simulink model "permanent_magnet_synchronous_machine"  (R2026b)
settings: Solver=VariableStepAuto
libraries: nesl_utility x24, fl_lib x1, pmsm_uvw_with_harmonics_lib x1
settings Model: Creator=dbagn  LastModifiedBy=d.bagnara

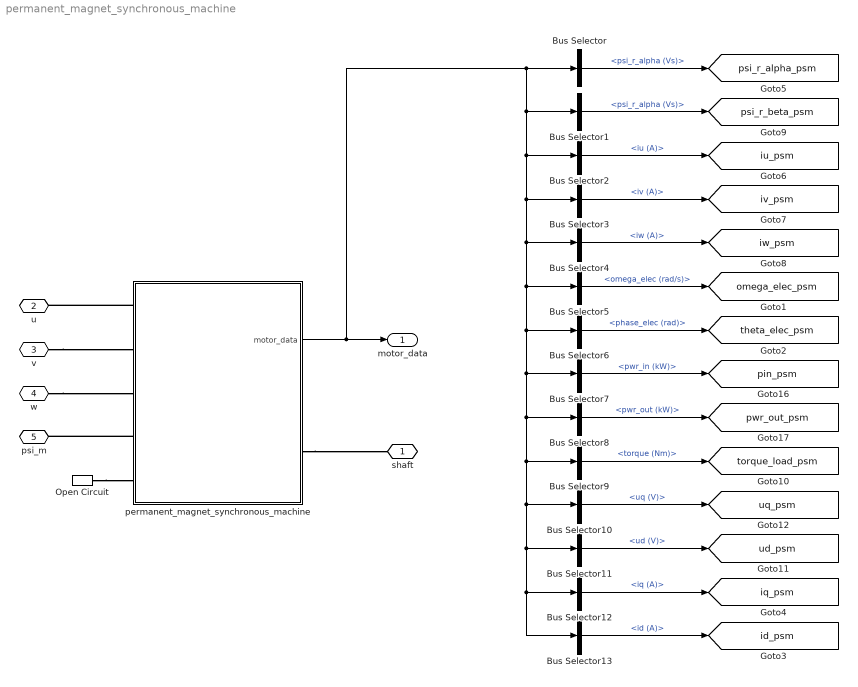
== system permanent_magnet_synchronous_machine ==
  Bus Selector : BusSelector  OutputSignals=psi_r_alpha (Vs)
  Bus Selector1 : BusSelector  OutputSignals=psi_r_alpha (Vs)
  Bus Selector10 : BusSelector  OutputSignals=uq (V)
  Bus Selector11 : BusSelector  OutputSignals=ud (V)
  Bus Selector12 : BusSelector  OutputSignals=iq (A)
  Bus Selector13 : BusSelector  OutputSignals=id (A)
  Bus Selector2 : BusSelector  OutputSignals=iu (A)
  Bus Selector3 : BusSelector  OutputSignals=iv (A)
  Bus Selector4 : BusSelector  OutputSignals=iw (A)
  Bus Selector5 : BusSelector  OutputSignals=omega_elec (rad/s)
  Bus Selector6 : BusSelector  OutputSignals=phase_elec (rad)
  Bus Selector7 : BusSelector  OutputSignals=pwr_in (kW)
  Bus Selector8 : BusSelector  OutputSignals=pwr_out (kW)
  Bus Selector9 : BusSelector  OutputSignals=torque (Nm)
  Open Circuit : fl_lib/Electrical/Electrical Elements/Open Circuit  v_specify=off  v_priority=None  v=0 V  v_nominal_specify=off  v_nominal_value=1  v_nominal_unit=V
  permanent_magnet_synchronous_machine : Subsystem  mask{pp=52, psi_m=3.85, Lmu=5e-6, La=4.6e-3, Lb=4.4e-3, Rs=31.5e-3, Jm=1968, b_linear=0, b_quadratic=0, h5_percent=0, h7_percent=0, psi_r_u_init=0, psi_r_v_init=0, psi_r_w_init=0, omega_init=0, phase_init=0, angle_error=0}
      mask prompts: pp "pole pairs"; psi_m "magnet flux - PsiM (Vs)"; Lmu "Leakage inductance - Lsigma (H)"; La "Phase self inductance - La (H)"; Lb "Phase mutual inductance - Lb (H)"; Rs "Phase resistance - Rs (Ohm)"; Jm "Shaft moment of inertia - Jm (kgm^2)"; b_linear "Linear viscosity - bm (Nms/rad)"; b_quadratic "Quadratic viscosity - bs (Nms^2/rad^2))"; h5_percent "Torque ripple H5 - (percent)"; h7_percent "Torque ripple H7 - (percent)"; psi_r_u_init "Rotor Flux init U - (Vs)"; psi_r_v_init "Rotor Flux init V - (Vs)"; psi_r_w_init "Rotor Flux init W - (Vs)"; omega_init "Rotor Speed init (rad/s)"; phase_init "Rotor Position init (rad)"; angle_error "Angle Error (rad)"
  shaft : PMIOPort  Side=Right
  u : PMIOPort  Port=2  Side=Left
  v : PMIOPort  Port=3  Side=Left
  w : PMIOPort  Port=4  Side=Left
  psi_m : PMIOPort  Port=5  Side=Left
  motor_data : Outport
  tag scope: id_psm=global, iq_psm=global, iu_psm=global, iv_psm=global, iw_psm=global, omega_elec_psm=global, pin_psm=global, psi_r_alpha_psm=global, psi_r_beta_psm=global, pwr_out_psm=global, theta_elec_psm=global, torque_load_psm=global, ud_psm=global, uq_psm=global
  wires:
  Bus Selector11/1 -> [ud_psm]  "<ud (V)>"
  Bus Selector9/1 -> [torque_load_psm]  "<torque (Nm)>"
  Bus Selector12/1 -> [iq_psm]  "<iq (A)>"
  Bus Selector13/1 -> [id_psm]  "<id (A)>"
  Bus Selector1/1 -> [psi_r_beta_psm]  "<psi_r_alpha (Vs)>"
  Bus Selector5/1 -> [omega_elec_psm]  "<omega_elec (rad/s)>"
  Bus Selector4/1 -> [iw_psm]  "<iw (A)>"
  Bus Selector2/1 -> [iu_psm]  "<iu (A)>"
  Bus Selector3/1 -> [iv_psm]  "<iv (A)>"
  Bus Selector6/1 -> [theta_elec_psm]  "<phase_elec (rad)>"
  permanent_magnet_synchronous_machine/1(motor_data) -> Bus Selector8/1, Bus Selector10/1, Bus Selector11/1, Bus Selector12/1, Bus Selector13/1, Bus Selector9/1, Bus Selector7/1, Bus Selector6/1, Bus Selector5/1, Bus Selector4/1, Bus Selector3/1, Bus Selector2/1, Bus Selector1/1, Bus Selector/1, motor_data/1
  Bus Selector7/1 -> [pin_psm]  "<pwr_in (kW)>"
  Bus Selector10/1 -> [uq_psm]  "<uq (V)>"
  Bus Selector/1 -> [psi_r_alpha_psm]  "<psi_r_alpha (Vs)>"
  Bus Selector8/1 -> [pwr_out_psm]  "<pwr_out (kW)>"
  connections:
  Open Circuit/LConn1 -- permanent_magnet_synchronous_machine/LConn5
  permanent_magnet_synchronous_machine/LConn4 -- psi_m/RConn1
  w/RConn1 -- permanent_magnet_synchronous_machine/LConn3
  permanent_magnet_synchronous_machine/RConn1 -- shaft/RConn1
  permanent_magnet_synchronous_machine/LConn1 -- u/RConn1
  v/RConn1 -- permanent_magnet_synchronous_machine/LConn2

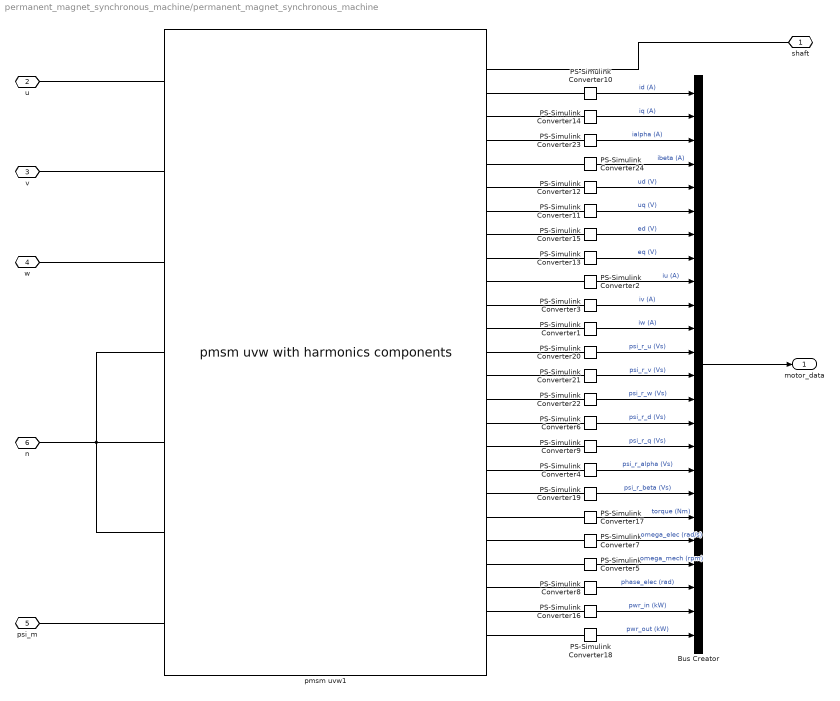
== system permanent_magnet_synchronous_machine/permanent_magnet_synchronous_machine ==
  Bus Creator : BusCreator  Inputs=24
  PS-Simulink Converter{1..3,10,14,23..24} (7 alike) : nesl_utility/PS-Simulink Converter  PhysicalDomain=network_engine_domain  SubClassName=ps_output  LeftPortType=input  RightPortType=output  PseudoPeriodic=off  Frequencies=[]  VectorFormat=1-D array  Unit=A  AffineConversion=off
  PS-Simulink Converter{11..13,15} (4 alike) : nesl_utility/PS-Simulink Converter  PhysicalDomain=network_engine_domain  SubClassName=ps_output  LeftPortType=input  RightPortType=output  PseudoPeriodic=off  Frequencies=[]  VectorFormat=1-D array  Unit=V  AffineConversion=off
  PS-Simulink Converter16 : nesl_utility/PS-Simulink Converter  PhysicalDomain=network_engine_domain  SubClassName=ps_output  LeftPortType=input  RightPortType=output  PseudoPeriodic=off  Frequencies=[]  VectorFormat=1-D array  Unit=kW  AffineConversion=off
  PS-Simulink Converter17 : nesl_utility/PS-Simulink Converter  PhysicalDomain=network_engine_domain  SubClassName=ps_output  LeftPortType=input  RightPortType=output  PseudoPeriodic=off  Frequencies=[]  VectorFormat=1-D array  Unit=N*m  AffineConversion=off
  PS-Simulink Converter18 : nesl_utility/PS-Simulink Converter  PhysicalDomain=network_engine_domain  SubClassName=ps_output  LeftPortType=input  RightPortType=output  PseudoPeriodic=off  Frequencies=[]  VectorFormat=1-D array  Unit=kW  AffineConversion=off
  PS-Simulink Converter{4,6,9,19..22} (7 alike) : nesl_utility/PS-Simulink Converter  PhysicalDomain=network_engine_domain  SubClassName=ps_output  LeftPortType=input  RightPortType=output  PseudoPeriodic=off  Frequencies=[]  VectorFormat=1-D array  Unit=V*s  AffineConversion=off
  PS-Simulink Converter5 : nesl_utility/PS-Simulink Converter  PhysicalDomain=network_engine_domain  SubClassName=ps_output  LeftPortType=input  RightPortType=output  PseudoPeriodic=off  Frequencies=[]  VectorFormat=1-D array  Unit=rpm  AffineConversion=off
  PS-Simulink Converter7 : nesl_utility/PS-Simulink Converter  PhysicalDomain=network_engine_domain  SubClassName=ps_output  LeftPortType=input  RightPortType=output  PseudoPeriodic=off  Frequencies=[]  VectorFormat=1-D array  Unit=rad/s  AffineConversion=off
  PS-Simulink Converter8 : nesl_utility/PS-Simulink Converter  PhysicalDomain=network_engine_domain  SubClassName=ps_output  LeftPortType=input  RightPortType=output  PseudoPeriodic=off  Frequencies=[]  VectorFormat=1-D array  Unit=rad  AffineConversion=off
  pmsm uvw1 : pmsm_uvw_with_harmonics_lib/pmsm uvw with harmonics components  number_poles=pp  psi_m_p=psi_m V*s  Lmu=Lmu H  La=La H  Lb=Lb H  Rs=Rs Ohm  J=Jm kg*m^2  b=b_linear N*m*s/rad  b_square=b_quadratic N*m*s^2/rad^2  h5=h5_percent percent  h7=h7_percent percent  angle_error=angle_error rad  omega_specify=on  omega_priority=High  omega=omega_init rad/s  omega_nominal_specify=off  omega_nominal_value=1  omega_nominal_unit=rad/s  theta_specify=on  theta_priority=High  theta=phase_init rad  theta_nominal_specify=off  theta_nominal_value=1  theta_nominal_unit=rad  iu_specify=off  iu_priority=None  iu=0 A  iu_nominal_specify=off  iu_nominal_value=1  iu_nominal_unit=A  iv_specify=off  iv_priority=None  iv=0 A  iv_nominal_specify=off  iv_nominal_value=1  iv_nominal_unit=A  iw_specify=off  iw_priority=None  iw=0 A  iw_nominal_specify=off  iw_nominal_value=1  iw_nominal_unit=A  id_specify=off  id_priority=None  id=0 A  id_nominal_specify=off  id_nominal_value=1  id_nominal_unit=A  iq_specify=off  iq_priority=None  iq=0 A  iq_nominal_specify=off  iq_nominal_value=1  iq_nominal_unit=A  ialpha_specify=off  ialpha_priority=None  ialpha=0 A  ialpha_nominal_specify=off  ialpha_nominal_value=1  ialpha_nominal_unit=A  ibeta_specify=off  ibeta_priority=None  ibeta=0 A  ibeta_nominal_specify=off  ibeta_nominal_value=1  ibeta_nominal_unit=A  uv_specify=off  uv_priority=None  uv=0 V  uv_nominal_specify=off  uv_nominal_value=1  uv_nominal_unit=V  uu_specify=off  uu_priority=None  uu=0 V  uu_nominal_specify=off  uu_nominal_value=1  uu_nominal_unit=V  uw_specify=off  uw_priority=None  uw=0 V  uw_nominal_specify=off  uw_nominal_value=1  uw_nominal_unit=V  ud_specify=off  ud_priority=None  ud=0 V  ud_nominal_specify=off  ud_nominal_value=1  ud_nominal_unit=V  uq_specify=off  uq_priority=None  uq=0 V  uq_nominal_specify=off  uq_nominal_value=1  uq_nominal_unit=V  psi_r_u_specify=on  psi_r_u_priority=High  psi_r_u=psi_r_u_init V*s  psi_r_u_nominal_specify=off  psi_r_u_nominal_value=1  psi_r_u_nominal_unit=V*s  psi_r_v_specify=on  psi_r_v_priority=High  psi_r_v=psi_r_v_init V*s  psi_r_v_nominal_specify=off  psi_r_v_nominal_value=1  psi_r_v_nominal_unit=V*s  psi_r_w_specify=on  psi_r_w_priority=High  psi_r_w=psi_r_w_init V*s  psi_r_w_nominal_specify=off  psi_r_w_nominal_value=1  psi_r_w_nominal_unit=V*s  psi_s_d_specify=off  psi_s_d_priority=None  psi_s_d=0.0 V*s  psi_s_d_nominal_specify=off  psi_s_d_nominal_value=1  psi_s_d_nominal_unit=V*s  psi_s_q_specify=off  psi_s_q_priority=None  psi_s_q=0.0 V*s  psi_s_q_nominal_specify=off  psi_s_q_nominal_value=1  psi_s_q_nominal_unit=V*s  psi_r_d_specify=off  psi_r_d_priority=High  psi_r_d=phi_m V*s  psi_r_d_nominal_specify=off  psi_r_d_nominal_value=1  psi_r_d_nominal_unit=V*s  psi_r_q_specify=off  psi_r_q_priority=High  psi_r_q=0.0 V*s  psi_r_q_nominal_specify=off  psi_r_q_nominal_value=1  psi_r_q_nominal_unit=V*s  psi_r_alpha_specify=off  psi_r_alpha_priority=High  psi_r_alpha=psi_m V*s  psi_r_alpha_nominal_specify=off  psi_r_alpha_nominal_value=1  psi_r_alpha_nominal_unit=V*s  psi_r_beta_specify=off  psi_r_beta_priority=High  psi_r_beta=0 V*s  psi_r_beta_nominal_specify=off  psi_r_beta_nominal_value=1  psi_r_beta_nominal_unit=V*s  psi_s_alpha_specify=off  psi_s_alpha_priority=None  psi_s_alpha=0.0 V*s  psi_s_alpha_nominal_specify=off  psi_s_alpha_nominal_value=1  psi_s_alpha_nominal_unit=V*s  psi_s_beta_specify=off  psi_s_beta_priority=None  psi_s_beta=0.0 V*s  psi_s_beta_nominal_specify=off  psi_s_beta_nominal_value=1  psi_s_beta_nominal_unit=V*s  tau_l_specify=off  tau_l_priority=None  tau_l=0 N*m  tau_l_nominal_specify=off  tau_l_nominal_value=1  tau_l_nominal_unit=N*m  tau_m_specify=off  tau_m_priority=None  tau_m=0 N*m  tau_m_nominal_specify=off  tau_m_nominal_value=1  tau_m_nominal_unit=N*m
  shaft : PMIOPort  Side=Right
  u : PMIOPort  Port=2  Side=Left
  v : PMIOPort  Port=3  Side=Left
  w : PMIOPort  Port=4  Side=Left
  psi_m : PMIOPort  Port=5  Side=Left
  n : PMIOPort  Port=6  Side=Left
  motor_data : Outport
  wires:
  PS-Simulink Converter14/1 -> Bus Creator/2  "iq (A)"
  Bus Creator/1 -> motor_data/1
  PS-Simulink Converter10/1 -> Bus Creator/1  "id (A)"
  PS-Simulink Converter18/1 -> Bus Creator/24  "pwr_out (kW)"
  PS-Simulink Converter16/1 -> Bus Creator/23  "pwr_in (kW)"
  PS-Simulink Converter8/1 -> Bus Creator/22  "phase_elec (rad)"
  PS-Simulink Converter5/1 -> Bus Creator/21  "omega_mech (rpm)"
  PS-Simulink Converter7/1 -> Bus Creator/20  "omega_elec (rad/s)"
  PS-Simulink Converter17/1 -> Bus Creator/19  "torque (Nm)"
  PS-Simulink Converter19/1 -> Bus Creator/18  "psi_r_beta (Vs)"
  PS-Simulink Converter4/1 -> Bus Creator/17  "psi_r_alpha (Vs)"
  PS-Simulink Converter12/1 -> Bus Creator/5  "ud (V)"
  PS-Simulink Converter11/1 -> Bus Creator/6  "uq (V)"
  PS-Simulink Converter15/1 -> Bus Creator/7  "ed (V)"
  PS-Simulink Converter13/1 -> Bus Creator/8  "eq (V)"
  PS-Simulink Converter2/1 -> Bus Creator/9  "iu (A)"
  PS-Simulink Converter23/1 -> Bus Creator/3  "ialpha (A)"
  PS-Simulink Converter24/1 -> Bus Creator/4  "ibeta (A)"
  PS-Simulink Converter9/1 -> Bus Creator/16  "psi_r_q (Vs)"
  PS-Simulink Converter6/1 -> Bus Creator/15  "psi_r_d (Vs)"
  PS-Simulink Converter22/1 -> Bus Creator/14  "psi_r_w (Vs)"
  PS-Simulink Converter21/1 -> Bus Creator/13  "psi_r_v (Vs)"
  PS-Simulink Converter20/1 -> Bus Creator/12  "psi_r_u (Vs)"
  PS-Simulink Converter1/1 -> Bus Creator/11  "iw (A)"
  PS-Simulink Converter3/1 -> Bus Creator/10  "iv (A)"
  connections:
  pmsm uvw1/LConn4 -- pmsm uvw1/LConn6 -- n/RConn1 -- pmsm uvw1/LConn5
  pmsm uvw1/RConn3 -- PS-Simulink Converter14/LConn1
  w/RConn1 -- pmsm uvw1/LConn3
  pmsm uvw1/LConn7 -- psi_m/RConn1
  pmsm uvw1/RConn2 -- PS-Simulink Converter10/LConn1
  pmsm uvw1/LConn1 -- u/RConn1
  pmsm uvw1/RConn1 -- shaft/RConn1
  v/RConn1 -- pmsm uvw1/LConn2
  pmsm uvw1/RConn25 -- PS-Simulink Converter18/LConn1
  pmsm uvw1/RConn24 -- PS-Simulink Converter16/LConn1
  pmsm uvw1/RConn23 -- PS-Simulink Converter8/LConn1
  PS-Simulink Converter5/LConn1 -- pmsm uvw1/RConn22
  PS-Simulink Converter7/LConn1 -- pmsm uvw1/RConn21
  PS-Simulink Converter17/LConn1 -- pmsm uvw1/RConn20
  pmsm uvw1/RConn6 -- PS-Simulink Converter12/LConn1
  pmsm uvw1/RConn8 -- PS-Simulink Converter15/LConn1
  pmsm uvw1/RConn7 -- PS-Simulink Converter11/LConn1
  pmsm uvw1/RConn9 -- PS-Simulink Converter13/LConn1
  PS-Simulink Converter2/LConn1 -- pmsm uvw1/RConn10
  pmsm uvw1/RConn4 -- PS-Simulink Converter23/LConn1
  PS-Simulink Converter24/LConn1 -- pmsm uvw1/RConn5
  pmsm uvw1/RConn19 -- PS-Simulink Converter19/LConn1
  pmsm uvw1/RConn18 -- PS-Simulink Converter4/LConn1
  pmsm uvw1/RConn17 -- PS-Simulink Converter9/LConn1
  pmsm uvw1/RConn16 -- PS-Simulink Converter6/LConn1
  pmsm uvw1/RConn15 -- PS-Simulink Converter22/LConn1
  pmsm uvw1/RConn14 -- PS-Simulink Converter21/LConn1
  pmsm uvw1/RConn13 -- PS-Simulink Converter20/LConn1
  pmsm uvw1/RConn12 -- PS-Simulink Converter1/LConn1
  pmsm uvw1/RConn11 -- PS-Simulink Converter3/LConn1
